simulink model "ASM_Traffic_A11"  (R2026a)
settings: Solver=ode1  StartTime=SIM.tstart.v  StopTime=SIM.tend.v  FixedStep=SIM.StepSize.v
PostLoadFcn:
  | if any(exist('dsrtsu_mdlpostloadfcn', 'file') ~= 0), dsrtsu_mdlpostloadfcn('Execute', bdroot); end
  | try, asm_mdl_postloadfcn(bdroot, 'UpdateModel', 3600); catch, disp(lasterr); end,
InitFcn:
  | , if any(exist('rtifpga_mdlclblib', 'file') ~= 0), rtifpga_mdlclblib('Init', bdroot); end,
  | , if any(exist('dsmpb_private', 'file') ~= 0), dsmpb_private('dsmpb_mdlclblib', 'Init', bdroot); end,
undefined symbols (not defined in the file): _to_, a0b2, ASM_BrakeHydraulics_DemoSystems, ASM_VehicleDynamics_DemoSystems, b98103fe8ad365046cd0, BrakeCircuit, controllerConfig, CPT, Crankshaft, DiscIntNeverNeededParam, dsmsi, FinalDriveAssembly, instance, MDL, ModeSignals, mu, Pos_BrakePedal_Maneuver, rad, RefSignals, s_to_rpm, SIM, SoftECU, Suspension, Tire, Transmission
libraries: ASM_Traffic_lib x135, simulink x98, ASM_Utils_lib x77, ASM_VehicleDynamics_lib x70, ASM_Environment_lib x22, dsmpblib x20, dsmsilib x15, MDLD_Utils_lib x10, ASM_BrakeHydraulics_lib x3, sl_discontinuities x2
(part 14 of 63)

== system ASM_Traffic_A11/Environment/Road/PlantModel ==
  UserInterface : Inport
  In : Inport  Port=2
  AMBIENT : ASM_Environment_lib/Environment/Road/AMBIENT  Tag=ASM_SUBCOMPONENT  Const_temperature=MDL.Environment.Ambient.Const_T  Const_pressure=MDL.Environment.Ambient.Const_p  ASMProperties=struct('Name','AMBIENT','Version','2.0','Library','ASM_Environment_lib')  ASMInstanceName=ambient  ASMInstanceID=1
  ASMSignalCollector : Subsystem
  BASIC_ROADS : ASM_Environment_lib/Environment/Road/BASIC_ROADS  Tag=ASM_SUBCOMPONENT  StepSize=SIM.StepSize  ASMProperties=struct('Name','BASIC_ROADS','Version','13.0','Library','ASM_Environment_lib')  ASMInstanceName=basic_roads  ASMInstanceID=1
  Bus Selector : BusSelector  OutputSignals=ModeSignals.Mode_Road[1NoRoad|2Straight|3Circle|4Road],MdlControl.Reset_VehicleStates[0|1],InitialVehStates.Pos_z_Vehicle_Rel_Init[m],MdlControl.Get_VehPos_Trigger[],Parameters.Curv_Road_Circle[1|m]
  Bus Selector10 : BusSelector  OutputSignals=ExternalModel.s_Preview[m]
  Bus Selector11 : BusSelector  OutputSignals=Slope_BasicRoad[%],Slope_Lateral_BasicRoad[deg],Fric_Coeff_CP_BasicRoad[:][],Sw_Tire_Parameter_Set_CP_BasicRoad[:][1|2|3|4]
  Bus Selector12 : BusSelector  OutputSignals=Sensor_Init_Ready[0Off|1On]
  Bus Selector13 : BusSelector  OutputSignals=ExternalModel.Active_CP_VehDyn_Trailer[]
  Bus Selector14 : BusSelector  OutputSignals=ExternalModel.Pos_CP_FL_CoorSys_E[x;y][m],ExternalModel.Pos_CP_FR_CoorSys_E[x;y][m],ExternalModel.Pos_CP_RL_CoorSys_E[x;y][m],ExternalModel.Pos_CP_RL2_CoorSys_E[x;y][m],ExternalModel.Pos_CP_RR_CoorSys_E[x;y][m],ExternalModel.Pos_CP_RR2_CoorSys_E[x;y][m],ExternalModel.Pos_CP_R2L_CoorSys_E[x;y][m],ExternalModel.Pos_CP_R2L2_CoorSys_E[x;y][m],ExternalModel.Pos_CP_R2R_CoorSys_E[x;y][m],ExternalModel.Pos_CP_R2R2_CoorSys_E[x;y][m],ExternalModel.Pos_CP_FL_Trailer_CoorSys_E[x;y][m],ExternalModel.Pos_CP_FL2_Trailer_CoorSys_E[x;y][m],ExternalModel.Pos_CP_FR_Trailer_CoorSys_E[x;y][m],ExternalModel.Pos_CP_FR2_Trailer_CoorSys_E[x;y][m],ExternalModel.Pos_CP_RL_Trailer_CoorSys_E[x;y][m],ExternalModel.Pos_CP_RL2_Trailer_CoorSys_E[x;y][m],ExternalModel.Pos_CP_RR_Trailer_CoorSys_E[x;y][m],ExternalModel.Pos_CP_RR2_Trailer_CoorSys_E[x;y][m],ExternalModel.Pos_CP_R2L_Trailer_CoorSys_E[x;y][m],ExternalModel.Pos_CP_R2L2_Trailer_CoorSys_E[x;y][m],ExternalModel.Pos_CP_R2R_Trailer_CoorSys_E[x;y][m],ExternalModel.Pos_CP_R2R2_Trailer_CoorSys_E[x;y][m],ExternalModel.Pos_CP_Front_CoorSys_E[x;y][m],ExternalModel.Pos_CP_Rear_CoorSys_E[x;y][m]  OutputAsBus=on
  Bus Selector15 : BusSelector  OutputSignals=ExternalModel.Angle_Vehicle_CoorSys_E[x;y;z][deg],ExternalModel.Pos_Vehicle_CoorSys_E[x;y;z][m]
  Bus Selector2 : BusSelector  OutputSignals=Sw_BasicRoad,Sw_RoadSelect[1_6]
  Bus Selector3 : BusSelector  OutputSignals=Route_Id_Fellows_Ref_Scheduler[],Direction_Fellows_Ref_Scheduler[-1|1],s_Fellows_Ref_Scheduler[m],d_Fellows_Ref_Scheduler[m],LaneIdx_Fellows_Ref_Scheduler[],RelativeLane_Mode_Fellows[0CenterLane|1PreferredLane],v_Lat_Fellows_Ref_Scheduler[m|s],ForceToRoad_Fellows_Ref_Scheduler[0|1],Flag_FellowUsed[0|1],Dist_Def_Trf[]
  Bus Selector4 : BusSelector  OutputSignals=Maneuver.Plant.ManeuverScheduler,Interface_In,Traffic.Plant.Traffic_Signals_toEnvironment,Sensors.Plant.Sensors_Common
  Bus Selector5 : BusSelector  OutputSignals=MdlControl.RoadControl[],InitialVehStates.Pos_z_Vehicle_Rel_Init[m],InitialVehStates.Angle_Yaw_Vehicle_Rel_Init[deg],InitialVehStates.Route_Id_Init[],InitialVehStates.Route_Direction_Init[],InitialVehStates.s_Vehicle_Init[m],InitialVehStates.d_Vehicle_Init[m],InitialVehStates.LaneIdx_Vehicle_Init[],RefSignals.d_Maneuver[m],RefSignals.LaneIdx_Maneuver[],ModeSignals.Mode_RelativeLane[0CenterLane|1PreferredLane],Parameters.v_Lat[m|s],ModeSignals.Mode_ForceToRoad[1Off|2On],RefSignals.Dist_Def_Maneuver[]
  Bus Selector7 : BusSelector  OutputSignals=ExternalModel.RotationMatrix_V_to_E[1x9]
  Bus Selector8 : BusSelector  OutputSignals=ExternalModel.v_x_Vehicle_CoG[km|h]
  Bus Selector9 : BusSelector  OutputSignals=Control.Interface_Mode[0Off|1ObjOnly|2ObjAndLanes],Control.Quadrant_Def_Mode[1Internal|2External],Control.Quadrant_Dim_x[m],Control.Quadrant_Dim_y[m]
  Const_4Road : Constant  Value=4
  Constant1 : Constant  Value=0
  Constant2 : Constant  Value=0
  Customize_UserSignals : Subsystem
  Demux : Demux  Outputs=3
  Demux1 : Demux  Outputs=3
  GPS_POSITION : ASM_Environment_lib/Environment/Road/GPS_POSITION  Tag=ASM_SUBCOMPONENT  ASMProperties=struct('Name','GPS_POSITION','Version','3.0','Library','ASM_Environment_lib')  ASMInstanceName=GPS_Position  ASMInstanceID=1
  Goto Tag Visibility : GotoTagVisibility  GotoTag=ASMBUS_Environment_BasicRoads
  Goto Tag Visibility1 : GotoTagVisibility  GotoTag=ASMBUS_Environment_StandardRoad
  Goto Tag Visibility2 : GotoTagVisibility  GotoTag=ASMBUS_Environment_LaneSensor_Dynamic_Parameters
  Goto Tag Visibility3 : GotoTagVisibility  GotoTag=ASMBUS_Environment_LaneSensor_Dynamic_Output
  Goto Tag Visibility4 : GotoTagVisibility  GotoTag=ASMBUS_Environment_Customized_UserSignals
  Goto Tag Visibility5 : GotoTagVisibility  GotoTag=ASMBUS_Environment_PosVehGPS
  Goto Tag Visibility6 : GotoTagVisibility  GotoTag=ASMBUS_Environment_Ambient
  Goto Tag Visibility7 : GotoTagVisibility  GotoTag=ASMBUS_Environment_Lane_Network
  LANESENSOR_DYNAMIC_OUTPUT : ASM_Environment_lib/Environment/Road/LANESENSOR_DYNAMIC_OUTPUT  Const_SensorPoints_OutputDimension=MDL.Environment.Road.LaneSensorDynamic_Output.Const_SensorPoints_OutputDimension  Const_MeasPoints_OutputDimension=MDL.Environment.Road.LaneSensorDynamic_Output.Const_MeasPoints_OutputDimension  Const_LanesLeft_OutputDimension=MDL.Environment.Road.LaneSensorDynamic_Output.Const_LanesLeft_OutputDimension  Const_LanesRight_OutputDimension=MDL.Environment.Road.LaneSensorDynamic_Output.Const_LanesRight_OutputDimension  ASMProperties=struct('Name','LANESENSOR_DYNAMIC_OUTPUT','Version','2.0','Library','ASM_Environment_lib')  ASMInstanceName=lanesensor_dynamic_output  ASMInstanceID=1
  LANESENSOR_DYNAMIC_PARAMETERS : ASM_Environment_lib/Environment/Road/LANESENSOR_DYNAMIC_PARAMETERS  Tag=ASM_SUBCOMPONENT  Sw_LaneSensor_Enable=MDL.Environment.Road.LaneSensorDynamic_Parameters.Sw_LaneSensor_Enable  Const_Dist_LaneSensor=MDL.Environment.Road.LaneSensorDynamic_Parameters.Const_Dist_LaneSensor  Sw_LaneSensor_Border_Mode=MDL.Environment.Road.LaneSensorDynamic_Parameters.Sw_LaneSensor_Border_Mode  Sw_LaneSensor_Junction_Enable=MDL.Environment.Road.LaneSensorDynamic_Parameters.Sw_LaneSensor_Junction_Enable  Const_NumLanes_Left=MDL.Environment.Road.LaneSensorDynamic_Parameters.Const_NumLanes_Left  Const_NumLanes_Right=MDL.Environment.Road.LaneSensorDynamic_Parameters.Const_NumLanes_Right  Sw_LaneSensor_MeasPoint_Enable=MDL.Environment.Road.LaneSensorDynamic_Parameters.Sw_LaneSensor_MeasPoint_Enable  Const_Pos_MeasPoint_1=MDL.Environment.Road.LaneSensorDynamic_Parameters.Const_Pos_MeasPoint_1  Const_Pos_MeasPoint_2=MDL.Environment.Road.LaneSensorDynamic_Parameters.Const_Pos_MeasPoint_2  Const_Pos_MeasPoint_3=MDL.Environment.Road.LaneSensorDynamic_Parameters.Const_Pos_MeasPoint_3  Const_Pos_MeasPoint_4=MDL.Environment.Road.LaneSensorDynamic_Parameters.Const_Pos_MeasPoint_4  ASMProperties=struct('Name','LANESENSOR_DYNAMIC_PARAMETERS','Version','1.0','Library','ASM_Environment_lib')  ASMInstanceName=lanesensor_dynamic_parameters  ASMInstanceID=1
  LANE_NETWORK : ASM_Environment_lib/Environment/Road/LANE_NETWORK  Tag=ASM_SUBCOMPONENT  LaneNetwork_ModelDesk=MDL.Environment.LaneNetwork.LaneNetwork_ModelDesk  LaneNetwork_2=MDL.Environment.LaneNetwork.LaneNetwork_2  LaneNetwork_3=MDL.Environment.LaneNetwork.LaneNetwork_3  LaneNetwork_4=MDL.Environment.LaneNetwork.LaneNetwork_4  LaneNetwork_5=MDL.Environment.LaneNetwork.LaneNetwork_5  LaneNetwork_6=MDL.Environment.LaneNetwork.LaneNetwork_6  Const_Quad_Dim_x=MDL.Environment.LaneNetwork.Const_Section_Dim_x  Const_Quad_Dim_y=MDL.Environment.LaneNetwork.Const_Section_Dim_y  Const_Max_Num_Lb_Quad=MDL.Environment.LaneNetwork.Const_Max_Num_Lb_Per_Section  Const_Max_Num_Pnts_Load=MDL.Environment.LaneNetwork.Const_Max_Num_Pnts_Per_Step  Const_Max_Num_Lanes_Load=MDL.Environment.LaneNetwork.Const_Max_Num_Lanes_Per_Step  Const_Max_Num_Lb_Free=MDL.Environment.LaneNetwork.Const_Max_Num_Lb_Free_Per_Step  Const_Max_Num_Lanes_Free=MDL.Environment.LaneNetwork.Const_Max_Num_Lanes_Free_Per_Step  ASMProperties=struct('Name','LANE_NETWORK','Version','5.0','Library','ASM_Environment_lib')  ASMInstanceName=lane_network  ASMInstanceID=1
  Mux : Mux  Inputs=2
  Mux1 : Mux  Inputs=2
  NoRoad : RelationalOperator  Operator===  OutDataTypeStr=boolean  InputSameDT=off
  Pos_CP_CoorsSys_E[:][x;y][m] : Subsystem
  Product1 : Product  RndMeth=Zero
  Product8 : Product  RndMeth=Zero
  ROAD : ASM_Environment_lib/Environment/Road/ROAD  Tag=ASM_SUBCOMPONENT  Road_ModelDesk=MDL.Environment.Road.Road_ModelDesk  Road_2=MDL.Environment.Road.Road_2  Road_3=MDL.Environment.Road.Road_3  Road_4=MDL.Environment.Road.Road_4  Road_5=MDL.Environment.Road.Road_5  Road_6=MDL.Environment.Road.Road_6  StepSize=SIM.StepSize  ASMProperties=struct('Name','ROAD','Version','32.0','Library','ASM_Environment_lib')  ASMInstanceName=road  ASMInstanceID=1
  Reload_Trigger : Subsystem
  Sat_RoadMode : Saturate  UpperLimit=4  LowerLimit=1
  Terminator{,1..19} (20 alike) : Terminator
  "[1x9]to[3x3]" : Reshape  OutputDimensionality=Customize  OutputDimensions=[3,3]
  ones26 : Constant  Value=ones(1,26)  OutDataTypeStr=double
  zero : Constant  Value=0
  ASMSignalBus : Outport  VectorParamsAs1DForOutWhenUnconnected=off
  tag scope: ASMBUS_Environment_Ambient=scoped, ASMBUS_Environment_BasicRoads=scoped, ASMBUS_Environment_Customized_UserSignals=scoped, ASMBUS_Environment_LaneSensor_Dynamic_Output=scoped, ASMBUS_Environment_LaneSensor_Dynamic_Parameters=scoped, ASMBUS_Environment_Lane_Network=scoped, ASMBUS_Environment_PosVehGPS=scoped, ASMBUS_Environment_StandardRoad=scoped
  wires:
  Bus Selector12/1 -> Reload_Trigger/1(Init_External_Additional[0Off|1On])  "<Sensor_Init_Ready[0Off|1On]>"
  Bus Selector4/4 -> Bus Selector12/1  "<Sensors_Common>"
  LANESENSOR_DYNAMIC_OUTPUT/2 -> Terminator7/1
  GPS_POSITION/2 -> Terminator6/1
  ROAD/10 -> Terminator3/1
  ROAD/8 -> Terminator2/1
  ROAD/6 -> Terminator1/1
  LANESENSOR_DYNAMIC_PARAMETERS/1 -> [ASMBUS_Environment_LaneSensor_Dynamic_Parameters]
  Bus Selector4/3 -> Bus Selector3/1, Bus Selector9/1  "<Traffic_Signals_toEnvironment>"
  GPS_POSITION/1 -> [ASMBUS_Environment_PosVehGPS]
  AMBIENT/2 -> Terminator4/1  "T_Ambient[degC]"
  Bus Selector10/1 -> Mux/2, BASIC_ROADS/6  "<s_Preview[m]>"
  Bus Selector4/1 -> Bus Selector/1, Bus Selector5/1  "<ManeuverScheduler>"
  Demux1/3 -> BASIC_ROADS/7, ROAD/19
  ROAD/4 -> Terminator11/1
  Bus Selector3/10 -> ROAD/32  "<Dist_Def_Trf[]>"
  In/1 -> Bus Selector4/1
  Bus Selector/2 -> BASIC_ROADS/2  "<Reset_VehicleStates[0|1]>"
  Bus Selector11/2 -> BASIC_ROADS/13  "<Slope_Lateral_BasicRoad[deg]>"
  Bus Selector7/1 -> "[1x9]to[3x3]"/1  "<RotationMatrix_V_to_E[1x9]>"
  Bus Selector9/1 -> LANE_NETWORK/3, Reload_Trigger/2(Interface_Mode[0Off|1ObjectsOnly|2ObjectsAndLanes])  "<Interface_Mode[0Off|1ObjOnly|2ObjAndLanes]>"
  Bus Selector11/4 -> BASIC_ROADS/15  "<Sw_Tire_Parameter_Set_CP_BasicRoad[:][1|2|3|4]>"
  Mux1/1 -> LANE_NETWORK/5
  Bus Selector5/12 -> ROAD/13  "<v_Lat[m|s]>"
  Bus Selector2/2 -> LANE_NETWORK/1, ROAD/1  "<Sw_RoadSelect[1_6]>"
  Bus Selector9/3 -> Mux1/1  "<Quadrant_Dim_x[m]>"
  Demux/2 -> BASIC_ROADS/9, LANESENSOR_DYNAMIC_PARAMETERS/2, GPS_POSITION/3, ROAD/18
  Bus Selector5/8 -> ROAD/9  "<LaneIdx_Vehicle_Init[]>"
  LANESENSOR_DYNAMIC_PARAMETERS/2 -> ROAD/33
  Bus Selector9/4 -> Mux1/2  "<Quadrant_Dim_y[m]>"
  ASMSignalCollector/1(Road_Signals) -> ASMSignalBus/1  "Plant"
  Bus Selector11/3 -> BASIC_ROADS/14  "<Fric_Coeff_CP_BasicRoad[:][]>"
  LANESENSOR_DYNAMIC_PARAMETERS/8 -> ROAD/39
  LANESENSOR_DYNAMIC_PARAMETERS/3 -> ROAD/34
  Bus Selector3/6 -> ROAD/28  "<RelativeLane_Mode_Fellows[0CenterLane|1PreferredLane]>"
  LANESENSOR_DYNAMIC_OUTPUT/1 -> [ASMBUS_Environment_LaneSensor_Dynamic_Output]
  LANESENSOR_DYNAMIC_PARAMETERS/7 -> ROAD/38
  Bus Selector3/7 -> ROAD/29  "<v_Lat_Fellows_Ref_Scheduler[m|s]>"
  Bus Selector2/1 -> Bus Selector11/1  "<Sw_BasicRoad>"
  Product1/1 -> ROAD/10
  Bus Selector3/9 -> ROAD/31  "<Flag_FellowUsed[0|1]>"
  Bus Selector5/14 -> ROAD/15  "<Dist_Def_Maneuver[]>"
  Bus Selector3/3 -> ROAD/25  "<s_Fellows_Ref_Scheduler[m]>"
  Product8/1 -> ROAD/11
  Bus Selector5/5 -> ROAD/6  "<Route_Direction_Init[]>"
  Bus Selector3/2 -> ROAD/24  "<Direction_Fellows_Ref_Scheduler[-1|1]>"
  Mux/1 -> ROAD/16
  Reload_Trigger/1(Ctrl_Reload[]) -> LANE_NETWORK/2
  ROAD/5 -> Terminator12/1
  Bus Selector/1 -> BASIC_ROADS/1, Sat_RoadMode/1  "<Mode_Road[1NoRoad|2Straight|3Circle|4Road]>"
  Bus Selector9/2 -> LANE_NETWORK/4  "<Quadrant_Def_Mode[1Internal|2External]>"
  BASIC_ROADS/5 -> Terminator15/1
  Bus Selector3/8 -> ROAD/30  "<ForceToRoad_Fellows_Ref_Scheduler[0|1]>"
  LANESENSOR_DYNAMIC_PARAMETERS/5 -> ROAD/36
  zero/1 -> Mux/1
  Const_4Road/1 -> NoRoad/2
  Bus Selector/3 -> BASIC_ROADS/3  "<Pos_z_Vehicle_Rel_Init[m]>"
  ones26/1 -> Product1/1, Product8/1
  BASIC_ROADS/1 -> [ASMBUS_Environment_BasicRoads]
  ROAD/3 -> Terminator10/1
  Sat_RoadMode/1 -> NoRoad/1
  ROAD/11 -> LANESENSOR_DYNAMIC_OUTPUT/1
  ROAD/7 -> Terminator/1
  ROAD/9 -> Customize_UserSignals/1(UserSignals_In)
  Bus Selector3/4 -> ROAD/26  "<d_Fellows_Ref_Scheduler[m]>"
  Bus Selector5/1 -> ROAD/2  "<RoadControl[]>"
  Bus Selector/5 -> BASIC_ROADS/5  "<Curv_Road_Circle[1|m]>"
  Bus Selector5/4 -> ROAD/5  "<Route_Id_Init[]>"
  Bus Selector/4 -> BASIC_ROADS/4  "<Get_VehPos_Trigger[]>"
  Bus Selector11/1 -> BASIC_ROADS/12  "<Slope_BasicRoad[%]>"
  Constant2/1 -> ROAD/22
  Bus Selector5/10 -> Product8/2  "<LaneIdx_Maneuver[]>"
  BASIC_ROADS/3 -> Terminator13/1
  Demux/1 -> ROAD/17, LANESENSOR_DYNAMIC_PARAMETERS/1, GPS_POSITION/2, BASIC_ROADS/8
  BASIC_ROADS/4 -> Terminator14/1
  LANESENSOR_DYNAMIC_PARAMETERS/4 -> ROAD/35
  Bus Selector5/11 -> ROAD/12  "<Mode_RelativeLane[0CenterLane|1PreferredLane]>"
  AMBIENT/3 -> Terminator16/1  "p_Ambient[Pa]"
  Bus Selector5/6 -> ROAD/7  "<s_Vehicle_Init[m]>"
  Constant1/1 -> ROAD/21
  Bus Selector5/7 -> ROAD/8  "<d_Vehicle_Init[m]>"
  LANESENSOR_DYNAMIC_PARAMETERS/6 -> ROAD/37
  NoRoad/1 -> ASMSignalCollector/1(SwitchRoad[0BasicRoad|1StandardRoad])
  Bus Selector3/1 -> ROAD/23  "<Route_Id_Fellows_Ref_Scheduler[]>"
  LANE_NETWORK/1 -> [ASMBUS_Environment_Lane_Network]
  ROAD/1 -> [ASMBUS_Environment_StandardRoad]
  Customize_UserSignals/1(ASMSignalBus) -> [ASMBUS_Environment_Customized_UserSignals]
  Bus Selector5/3 -> ROAD/4  "<Angle_Yaw_Vehicle_Rel_Init[deg]>"
  Bus Selector5/2 -> ROAD/3  "<Pos_z_Vehicle_Rel_Init[m]>"
  Bus Selector5/13 -> ROAD/14  "<Mode_ForceToRoad[1Off|2On]>"
  Bus Selector5/9 -> Product1/2  "<d_Maneuver[m]>"
  AMBIENT/1 -> [ASMBUS_Environment_Ambient]
  UserInterface/1 -> Bus Selector2/1
  Customize_UserSignals/2(UserSignals_Customized) -> GPS_POSITION/1
  ROAD/2 -> Terminator5/1
  BASIC_ROADS/2 -> Terminator8/1
  Bus Selector3/5 -> ROAD/27  "<LaneIdx_Fellows_Ref_Scheduler[]>"
  "[1x9]to[3x3]"/1 -> LANESENSOR_DYNAMIC_PARAMETERS/3
  LANE_NETWORK/2 -> Terminator9/1  "LaneNetwork_Data[]"
  Bus Selector4/2 -> Bus Selector8/1, Bus Selector10/1, Bus Selector15/1, Bus Selector14/1, Bus Selector13/1, Bus Selector7/1  "<Interface_In>"
  Bus Selector14/1 -> Pos_CP_CoorsSys_E[:][x;y][m]/1(Pos_CP[x;y][m])
  Bus Selector13/1 -> Pos_CP_CoorsSys_E[:][x;y][m]/2(Active_CP_VehDyn_Trailer[])  "<Active_CP_VehDyn_Trailer[]>"
  Pos_CP_CoorsSys_E[:][x;y][m]/1(Pos_CP_CoorsSys_E[:][x;y][m]) -> ROAD/20, BASIC_ROADS/10
  Bus Selector8/1 -> BASIC_ROADS/11  "<v_x_Vehicle_CoG[km|h]>"
  Demux/3 -> Terminator17/1
  Bus Selector15/2 -> Demux/1  "<Pos_Vehicle_CoorSys_E[x;y;z][m]>"
  Bus Selector15/1 -> Demux1/1  "<Angle_Vehicle_CoorSys_E[x;y;z][deg]>"
  Demux1/1 -> Terminator18/1
  Demux1/2 -> Terminator19/1

== system ASM_Traffic_A11/Environment/Road/UserInterface ==
  note: Road
  Interface_In : Inport
  In : Inport  Port=2
  ASMSignalBus_Plant : Subsystem
  DISP_Plant : Subsystem
  PAR_Plant : Subsystem
  Out : Outport  VectorParamsAs1DForOutWhenUnconnected=off
  wires:
  PAR_Plant/1(Out) -> Out/1
  Interface_In/1 -> PAR_Plant/1(Interface_In)
  In/1 -> ASMSignalBus_Plant/1(In), DISP_Plant/1(In)

== system ASM_Traffic_A11/Environment/Sensors/PlantModel ==
  UserInterface : Inport
  In : Inport  Port=2
  ASMSignalCollector : Subsystem
  Bus Selector7 : BusSelector  OutputSignals=Traffic,Interface_In,Road,Maneuver,Road.UserInterface.Objects_DataStreams[]
  Collision_Sensor : Subsystem
  Line_Sensor : Subsystem
  Object_Sensor_2D : Subsystem
  Object_Sensor_3D : Subsystem
  SensorsGotoTagVisiblity : GotoTagVisibility  GotoTag=ASMBUS_Environment_Trafffic_Sensors_Object_Sensor_3D
  SensorsGotoTagVisiblity1 : GotoTagVisibility  GotoTag=ASMBUS_Environment_Traffic_Sensors_Object_Sensor_2D
  SensorsGotoTagVisiblity2 : GotoTagVisibility  GotoTag=ASMBUS_Environment_Traffic_Sensors_Traffic_Sign_Sensor_dyn
  SensorsGotoTagVisiblity3 : GotoTagVisibility  GotoTag=ASMBUS_Environment_Traffic_Sensors_Line_Sensor
  SensorsGotoTagVisiblity4 : GotoTagVisibility  GotoTag=ASMBUS_Environment_Traffic_Sensors_Collision_Sensor
  SensorsGotoTagVisiblity5 : GotoTagVisibility  GotoTag=ASMBUS_Environment_Traffic_Sensors_Common
  Sensors_Common_Signals : Subsystem
  Terminator{,1..5} (6 alike) : Terminator
  Traffic_Sign_Sensor : Subsystem
  ASMSignalBus : Outport  VectorParamsAs1DForOutWhenUnconnected=off
  tag scope: ASMBUS_Environment_Traffic_Sensors_Common=scoped
  wires:
  In/1 -> Sensors_Common_Signals/1(In), Bus Selector7/1
  Sensors_Common_Signals/1(ASMSignalBus) -> [ASMBUS_Environment_Traffic_Sensors_Common]
  Object_Sensor_3D/2(Init_Ready[0Off|1On]) -> Object_Sensor_2D/1(Enable_Init[0Off|1On])
  Sensors_Common_Signals/4(Enable_Sensor_Scheduling[0Off|1On]) -> Line_Sensor/1(Enable[0Off|1On])
  Object_Sensor_2D/2(Init_Ready[0Off|1On]) -> Sensors_Common_Signals/2(Init_Ready[0Off|1On]), Collision_Sensor/1(Enable_Init[0Off|1On])
  Sensors_Common_Signals/2(Enable_Init[0Off|1On]) -> Object_Sensor_3D/1(Enable_Init[0Off|1On])
  Sensors_Common_Signals/3(Enable_Sensor_Scheduling_By_Init_Ready[0Off|1On]) -> Object_Sensor_2D/2(Enable[0Off|1On]), Collision_Sensor/2(Enable[0Off|1On]), Object_Sensor_3D/2(Enable[0Off|1On])
  Object_Sensor_3D/1(Sensor_Signals) -> Terminator5/1  "Object_Sensor_3D"
  Object_Sensor_2D/1(Sensor_Signals) -> Terminator1/1  "Object_Sensor_2D"
  Traffic_Sign_Sensor/1(Sensor_Signals) -> Terminator2/1  "Traffic_Sign_Sensor"
  Line_Sensor/1(Sensor_Signals) -> Terminator3/1  "Line_Sensor"
  Collision_Sensor/1(Sensor_Signals) -> Terminator4/1  "Collision_Sensor"
  ASMSignalCollector/1(Sensors) -> ASMSignalBus/1  "Plant"
  UserInterface/1 -> Terminator/1
  Bus Selector7/5 -> Traffic_Sign_Sensor/4(Objects_DataStream_Signals)  "<Objects_DataStreams[]>"
  Bus Selector7/4 -> Collision_Sensor/6(Maneuver_Signals), Line_Sensor/4(Maneuver_Signals)  "<Maneuver>"
  Bus Selector7/3 -> Collision_Sensor/5(Road_Signals), Line_Sensor/3(Road_Signals), Traffic_Sign_Sensor/3(Road_Signals), Object_Sensor_2D/5(Road_Signals), Object_Sensor_3D/5(Road_Signals)  "<Road>"
  Bus Selector7/1 -> Collision_Sensor/3(Traffic_Signals), Traffic_Sign_Sensor/2(Traffic_Signals), Object_Sensor_2D/3(Traffic_Signals), Object_Sensor_3D/3(Traffic_Signals)  "<Traffic>"
  Bus Selector7/2 -> Collision_Sensor/4(Interface_In), Line_Sensor/2(Interface_In), Traffic_Sign_Sensor/1(Interface_In), Object_Sensor_2D/4(Interface_In), Object_Sensor_3D/4(Interface_In)  "<Interface_In>"
  Sensors_Common_Signals/5(Sensor_Time_Base[s]) -> Object_Sensor_3D/6(Sensor_Time_Base[s])

== system ASM_Traffic_A11/Environment/Sensors/UserInterface ==
  note: Sensors
  In : Inport
  ASMSignalBus_Plant : Subsystem
  DISP_Plant : Subsystem
  PAR_Plant : Subsystem
  Out : Outport  VectorParamsAs1DForOutWhenUnconnected=off
  wires:
  PAR_Plant/1(Out) -> Out/1
  In/1 -> ASMSignalBus_Plant/1(In), PAR_Plant/1(In), DISP_Plant/1(In)

== system ASM_Traffic_A11/Environment/SignalInterface/ASMSignalInterface ==
  ASMSignalBus : Inport
  Enable : EnablePort
  signal_structure : Subsystem
  wires:
  ASMSignalBus/1 -> signal_structure/1(ASMSignalBus)

== system ASM_Traffic_A11/Environment/SignalInterface/ExternalOutports ==
  In1 : Inport
  Enable : EnablePort
  Environment : dsmpblib/Data Outport  Tag=ASM_MPB  Priority=-10000
      settings: SourceProductName=dSPACE Model Interface Package for Simulink (MIPS)
  Select_Outport_Signals : Subsystem
  wires:
  In1/1 -> Select_Outport_Signals/1(ASMSignalBus)
  Select_Outport_Signals/5(Sensors) -> Environment/5
  Select_Outport_Signals/4(GroundTruth) -> Environment/4
  Select_Outport_Signals/3(Traffic) -> Environment/3
  Select_Outport_Signals/2(Road) -> Environment/2
  Select_Outport_Signals/1(Maneuver) -> Environment/1

== system ASM_Traffic_A11/Environment/SignalInterface/Reduce_ASMSignalBus ==
  ASMSignalBus : Inport
  Bus Creator : BusCreator  Inputs=5
  Bus Creator1 : BusCreator  Inputs=8
  Bus Creator2 : BusCreator  Inputs=8
  Bus Creator3 : BusCreator  Inputs=6
  Bus Creator4 : BusCreator  Inputs=5
  Bus Selector : BusSelector  OutputSignals=Maneuver,Road,Traffic,GroundTruth,Sensors
  Bus Selector1 : BusSelector  OutputSignals=Parameter,SensorIndex,Info,SensorOutput,SensorTimeStamp,RadarEffects,CustomPoints,ObjectData
  Bus Selector2 : BusSelector  OutputSignals=Parameter,SensorIndex,Info,SensorOutput,SensorTimeStamp,RadarEffects,CustomPoints,ObjectData
  Bus Selector3 : BusSelector  OutputSignals=Parameters,SensorIndex,SensorStatus,SensorOutput,Info,ObjectData
  Bus Selector4 : BusSelector  OutputSignals=Collision_Sensor,TrafficSign_Sensor_Dyn,Object_Sensor_3D.Sensor_1_Front_Long,Object_Sensor_3D.Sensor_2_Front_Mid,Object_Sensor_2D.Sensor_1_Front
  ASMSignalBus_Reduced : Outport  VectorParamsAs1DForOutWhenUnconnected=off
  wires:
  Bus Selector3/6 -> Bus Creator3/6  "<ObjectData>"
  Bus Selector3/5 -> Bus Creator3/5  "<Info>"
  Bus Selector3/4 -> Bus Creator3/4  "<SensorOutput>"
  Bus Selector3/3 -> Bus Creator3/3  "<SensorStatus>"
  Bus Selector3/2 -> Bus Creator3/2  "<SensorIndex>"
  Bus Selector3/1 -> Bus Creator3/1  "<Parameters>"
  Bus Creator3/1 -> Bus Creator4/5  "Object_Sensor_2D_1"
  Bus Selector4/5 -> Bus Selector3/1  "<Sensor_1_Front>"
  Bus Selector4/4 -> Bus Selector2/1  "<Sensor_2_Front_Mid>"
  Bus Selector2/1 -> Bus Creator2/1  "<Parameter>"
  Bus Selector2/2 -> Bus Creator2/2  "<SensorIndex>"
  Bus Selector2/3 -> Bus Creator2/3  "<Info>"
  Bus Selector2/4 -> Bus Creator2/4  "<SensorOutput>"
  Bus Selector2/5 -> Bus Creator2/5  "<SensorTimeStamp>"
  Bus Selector2/6 -> Bus Creator2/6  "<RadarEffects>"
  Bus Selector2/7 -> Bus Creator2/7  "<CustomPoints>"
  Bus Selector2/8 -> Bus Creator2/8  "<ObjectData>"
  Bus Creator2/1 -> Bus Creator4/4  "Object_Sensor_3D_2"
  Bus Creator1/1 -> Bus Creator4/3  "Object_Sensor_3D_1"
  Bus Selector1/8 -> Bus Creator1/8  "<ObjectData>"
  Bus Selector1/7 -> Bus Creator1/7  "<CustomPoints>"
  Bus Selector1/6 -> Bus Creator1/6  "<RadarEffects>"
  Bus Selector1/5 -> Bus Creator1/5  "<SensorTimeStamp>"
  Bus Selector1/4 -> Bus Creator1/4  "<SensorOutput>"
  Bus Selector1/3 -> Bus Creator1/3  "<Info>"
  Bus Selector1/2 -> Bus Creator1/2  "<SensorIndex>"
  Bus Selector1/1 -> Bus Creator1/1  "<Parameter>"
  Bus Selector4/3 -> Bus Selector1/1  "<Sensor_1_Front_Long>"
  Bus Selector4/2 -> Bus Creator4/2  "<TrafficSign_Sensor_Dyn>"
  Bus Selector/2 -> Bus Creator/2  "<Road>"
  Bus Selector/3 -> Bus Creator/3  "<Traffic>"
  Bus Creator/1 -> ASMSignalBus_Reduced/1
  Bus Selector/1 -> Bus Creator/1  "<Maneuver>"
  ASMSignalBus/1 -> Bus Selector/1
  Bus Selector/4 -> Bus Creator/4  "<GroundTruth>"
  Bus Selector/5 -> Bus Selector4/1  "<Sensors>"
  Bus Selector4/1 -> Bus Creator4/1  "<Collision_Sensor>"
  Bus Creator4/1 -> Bus Creator/5  "Sensors"

== system ASM_Traffic_A11/Environment/Traffic/PlantModel ==
  UserInterface : Inport
  In : Inport  Port=2
  Bus Creator2 : BusCreator  Inputs=4
  Bus Selector1 : BusSelector  OutputSignals=FellowSignalLabels
  Bus Selector16 : BusSelector  OutputSignals=Road,Maneuver,Interface_In,Traffic.Plant.ObjectParameters,Road.UserInterface.Objects_DataStreams[],Traffic,GroundTruth,Sensors
  FellowMovement : Subsystem
  Merge_Signals_toEnvironment : Subsystem
  ObjectParameters : Subsystem
  V2X : Subsystem
  ASMSignalBus : Outport  VectorParamsAs1DForOutWhenUnconnected=off
  wires:
  ObjectParameters/1(Objects_Signals) -> Bus Creator2/3
  Bus Selector1/1 -> Bus Creator2/2  "<FellowSignalLabels>"
  FellowMovement/1(FellowMovement_Signals) -> Bus Selector1/1, Merge_Signals_toEnvironment/1(Traffic_Signals)
  Bus Selector16/7 -> Merge_Signals_toEnvironment/2(GroundTruth_Interface)  "<GroundTruth>"
  Bus Creator2/1 -> ASMSignalBus/1  "Plant"
  Bus Selector16/5 -> FellowMovement/6(Object_DataStreams)  "<Objects_DataStreams[]>"
  In/1 -> Bus Selector16/1
  Bus Selector16/3 -> FellowMovement/4(Interface_In)  "<Interface_In>"
  UserInterface/1 -> V2X/3(UserInterface), FellowMovement/1(UserInterface)
  Merge_Signals_toEnvironment/1(Signals_toEnvironment) -> Bus Creator2/1
  Bus Selector16/2 -> V2X/2(Maneuver_Signals), ObjectParameters/2(Maneuver_Signals), FellowMovement/3(Maneuver_Signals)  "<Maneuver>"
  Bus Selector16/1 -> ObjectParameters/1(Road_Signals), V2X/1(Road_Signals), FellowMovement/2(Road_Signals)  "<Road>"
  Bus Selector16/4 -> FellowMovement/5(ObjectParameters_Signals)  "<ObjectParameters>"
  V2X/1(V2X_Signals) -> Bus Creator2/4
  Bus Selector16/6 -> FellowMovement/7(Traffic_Signals)  "<Traffic>"
  Bus Selector16/8 -> ObjectParameters/3(Sensor_Signals)  "<Sensors>"

== system ASM_Traffic_A11/Environment/Traffic/UserInterface ==
  note: Traffic
  In : Inport
  ASMSignalBus_Plant : Subsystem
  DISP_Plant : Subsystem
  PAR_Plant : Subsystem
  Out : Outport  VectorParamsAs1DForOutWhenUnconnected=off
  wires:
  PAR_Plant/1(Out) -> Out/1
  In/1 -> ASMSignalBus_Plant/1(In), DISP_Plant/1(In)

== system ASM_Traffic_A11/VehicleDynamics/Control/SoftECU_Brake ==
  note: -------------
  note: Control
  note: -------------
  note: -------------
  note: -------------
  note: Inport colors:
  note: User Interface
  note: Plant
  note: External Signals
  UserInterface : Inport
  Interface_In : Inport  Port=2
  Plant : Inport  Port=3
  Brake_Topology_Switch : Subsystem
  Bus Creator : BusCreator  Inputs=5
  Bus Selector1 : BusSelector  OutputSignals=ExternalModel.Enable_Trq_Brake_Extern[0|1],ExternalModel.Trq_Brake_Request_Extern[Nm],ExternalModel.Trq_Request_Brake[Nm]
  Bus Selector10 : BusSelector  OutputSignals=ExternalModel.Vehicle_Topology[-2|-1|0|2],ExternalModel.Trq_Eff_Engine[Nm],ExternalModel.Trq_EM_Front[Nm]
  Bus Selector2 : BusSelector  OutputSignals=VehicleDynamics.Brake.BrakeDisc.Const_BrakeDiscFactor.Const_BrakeDiscFactor_FL[m3],VehicleDynamics.Brake.BrakeDisc.Const_BrakeDiscFactor.Const_BrakeDiscFactor_FR[m3],VehicleDynamics.Brake.BrakeDisc.Const_BrakeDiscFactor.Const_BrakeDiscFactor_RL[m3],VehicleDynamics.Brake.BrakeDisc.Const_BrakeDiscFactor.Const_BrakeDiscFactor_RR[m3],VehicleDynamics.Brake.MasterBrakeCylinder.ActiveBrakeCylinder.p[bar],VehicleDynamics.VehicleMovement.Velocities.Vehicle.Linear.v_Vehicle_CoG[x;y;z][km|h].v_x_Vehicle_CoG[km|h],VehicleDynamics.VehicleMovement.Velocities.Vehicle.Linear.v_Vehicle_CoG[x;y;z][km|h].v_y_Vehicle_CoG[km|h],VehicleDynamics.VehicleMovement.Accelerations.VehicleCoG.Linear.a_Vehicle_CoG[x;y;z][m|s2].a_y_Vehicle_CoG[m|s2],VehicleDynamics.VehicleMovement.Velocities.Vehicle.Angular.w_Vehicle_CoG[x;y;z][deg|s].YawRate_Vehicle_CoG[deg|s],VehicleDynamics.Wheel.WheelSpeed2.omega_Wheel[FL;FR;RL;RR][rad|s],VehicleDynamics.Steering.Angle_SteeringWheel[deg],VehicleDynamics.Steering.i_Steering_Mean[],VehicleDynamics.Suspension.SuspensionRear.RelativePositionRear.Pos_Wheel[RL;RR][x;y;z][m].Pos_RL_Wheel[x;y;z][m],VehicleDynamics.Suspension.SuspensionFront.RelativePositionFront.Pos_Wheel[FL;FR][x;y;z][m].Pos_FL_Wheel[x;y;z][m],VehicleDynamics.Tire.r_Dyn_Tire[FL;FR;RL;RR][m]
  Bus Selector3 : BusSelector  OutputSignals=ESP_Switches
  Bus Selector4 : BusSelector  OutputSignals=ExternalModel.Reset_VehicleStates[0|1],ExternalModel.ECU_Commands[],ExternalModel.Pos_AccPedal[%],ExternalModel.Pos_BrakePedal[%]
  Engine_Topology_Switch : Subsystem
  HideBusFeedback : DataTypeConversion  SaturateOnIntegerOverflow=off  RndMeth=Floor
  HideBusFeedback1 : DataTypeConversion  SaturateOnIntegerOverflow=off  RndMeth=Floor
  Map_Inputs : Subsystem
  ModelDesk_MC_ID_SoftECU : ASM_Utils_lib/ModelDeskInterface/ModelDesk_MC  Tag=ASM_MAINCOMPONENT  Editable=off  MainComponent=SoftECU
  Mux1 : Mux
  OpenBrakeSoftECU : ASM_Utils_lib/Miscellaneous/OpenSystem  popupLibBlk=<select here>  popupTargetDemo=<select here>  Demosystem=BrakeHydraulics_SoftECU  variantLib=ASM_BrakeHydraulics_DemoSystems/SoftECU
  Soft_ECU_Brake : Subsystem  Tag=BrakeHydraulics_SoftECU
  ASMSignalBus : Outport  VectorParamsAs1DForOutWhenUnconnected=off
  Out : Outport  Port=2  VectorParamsAs1DForOutWhenUnconnected=off
  wires:
  UserInterface/1 -> Bus Selector3/1
  Map_Inputs/2(Sw_ASR[0Off|1On]) -> Soft_ECU_Brake/7(Sw_ASR[0Off|1On])
  Map_Inputs/1(Sw_ESP[0Off|1ABS|ESP]) -> Soft_ECU_Brake/6(Sw_ESP[0Off|1ABS|2ESP])
  HideBusFeedback1/1 -> Soft_ECU_Brake/3(Trq_Request_Extern[Nm])
  HideBusFeedback/1 -> Soft_ECU_Brake/1(State_Brake_Without_BrkPedal[0|1]), Soft_ECU_Brake/2(Enable_Trq_Extern[0|1])
  Bus Creator/1 -> Out/1
  Soft_ECU_Brake/2(Enable_p_Brake_Desired[0|1]) -> Bus Creator/1
  Soft_ECU_Brake/3(p_Brake_Desired[bar]) -> Bus Creator/2
  Soft_ECU_Brake/4(ECU_Mode[0None|1ABS|2ESP|3ASR]) -> Bus Creator/3
  Soft_ECU_Brake/5(Valves) -> Bus Creator/4
  Soft_ECU_Brake/6(Trq_Intervention) -> Bus Creator/5
  Bus Selector1/2 -> Brake_Topology_Switch/2(Trq_Brake_Request_Extern[Nm])  "<Trq_Brake_Request_Extern[Nm]>"
  Bus Selector1/1 -> Brake_Topology_Switch/1(Enable_Trq_Brake_Extern[0|1])  "<Enable_Trq_Brake_Extern[0|1]>"
  Interface_In/1 -> Bus Selector1/1, Bus Selector10/1, Bus Selector4/1
  Soft_ECU_Brake/1(ASMSignalBus) -> ASMSignalBus/1
  Bus Selector4/2 -> Map_Inputs/3(ECU_Commands[])  "<ECU_Commands[]>"
  Bus Selector4/1 -> Soft_ECU_Brake/5(Reset[]), Map_Inputs/1(Reset[0|1])  "<Reset_VehicleStates[0|1]>"
  Bus Selector4/3 -> Soft_ECU_Brake/17(Pos_AccPedal[%])  "<Pos_AccPedal[%]>"
  Bus Selector4/4 -> Soft_ECU_Brake/18(Pos_BrakePedal[%])  "<Pos_BrakePedal[%]>"
  Bus Selector3/1 -> Map_Inputs/2(Switches_ESP_User)  "<ESP_Switches>"
  Plant/1 -> Bus Selector2/1
  Bus Selector2/1 -> Mux1/1  "<Const_BrakeDiscFactor_FL[m3]>"
  Bus Selector2/2 -> Mux1/2  "<Const_BrakeDiscFactor_FR[m3]>"
  Bus Selector2/3 -> Mux1/3  "<Const_BrakeDiscFactor_RL[m3]>"
  Bus Selector2/4 -> Mux1/4  "<Const_BrakeDiscFactor_RR[m3]>"
  Mux1/1 -> Soft_ECU_Brake/4(Const_BrakeDiscFactor[FL;FR;RL;RR][m3])
  Bus Selector2/5 -> Soft_ECU_Brake/9(p_MasterBrakeCyl[bar])  "<p[bar]>"
  Bus Selector2/6 -> Soft_ECU_Brake/10(v_x_Vehicle_CoG[km|h])  "<v_x_Vehicle_CoG[km|h]>"
  Bus Selector2/7 -> Soft_ECU_Brake/11(v_y_Vehicle_CoG[km|h])  "<v_y_Vehicle_CoG[km|h]>"
  Bus Selector2/8 -> Soft_ECU_Brake/12(a_y_Vehicle_CoG[m|s2])  "<a_y_Vehicle_CoG[m|s2]>"
  Bus Selector2/9 -> Soft_ECU_Brake/13(YawRate_Vehicle_CoG[deg|s])  "<YawRate_Vehicle_CoG[deg|s]>"
  Bus Selector2/10 -> Soft_ECU_Brake/14(WheelSpeed[FL;FR;RL;RR][rad|s])  "<omega_Wheel[FL;FR;RL;RR][rad|s]>"
  Bus Selector2/11 -> Soft_ECU_Brake/15(Angle_SteeringWheel[deg])  "<Angle_SteeringWheel[deg]>"
  Bus Selector2/12 -> Soft_ECU_Brake/16(i_Steering_Mean[])  "<i_Steering_Mean[]>"
  Bus Selector2/13 -> Soft_ECU_Brake/19(Pos_RL_Wheel[x;y;z][m])  "<Pos_RL_Wheel[x;y;z][m]>"
  Bus Selector2/14 -> Soft_ECU_Brake/20(Pos_FL_Wheel[x;y;z][m])  "<Pos_FL_Wheel[x;y;z][m]>"
  Bus Selector2/15 -> Soft_ECU_Brake/21(r_Tire[m])  "<r_Dyn_Tire[FL;FR;RL;RR][m]>"
  Bus Selector1/3 -> Brake_Topology_Switch/3(Trq_Request_Brake[Nm])  "<Trq_Request_Brake[Nm]>"
  Brake_Topology_Switch/1(Enable_Trq_Extern[0|1]) -> HideBusFeedback/1
  Brake_Topology_Switch/2(Trq_Request_Extern[Nm]) -> HideBusFeedback1/1
  Engine_Topology_Switch/1(Trq[Nm]) -> Soft_ECU_Brake/8(Trq_Eff_Engine[Nm])
  Bus Selector10/1 -> Brake_Topology_Switch/4(Vehicle_Topology[-2|-1|0|2]), Engine_Topology_Switch/1(Vehicle_Topology[-2|-1|0|2])  "<Vehicle_Topology[-2|-1|0|2]>"
  Bus Selector10/2 -> Engine_Topology_Switch/2(Trq_Eff_Engine[Nm])  "<Trq_Eff_Engine[Nm]>"
  Bus Selector10/3 -> Engine_Topology_Switch/3(Trq_EM_Front[Nm])  "<Trq_EM_Front[Nm]>"

== system ASM_Traffic_A11/VehicleDynamics/Control/SoftECU_Steering ==
  note: -------------
  note: Control
  note: -------------
  note: -------------
  note: -------------
  note: Inport colors:
  note: User Interface
  note: Plant
  note: External Signals
  UserInterface : Inport
  Interface_In : Inport  Port=2
  Plant : Inport  Port=3
  Bus Creator : BusCreator  Inputs=1
  Bus Selector : BusSelector  OutputSignals=ExternalModel.Reset_VehicleStates[0|1],ExternalModel.Sw_Ignition[0Off|1On]
  Bus Selector1 : BusSelector  OutputSignals=VehicleDynamics.Steering.ForcesAndTorques.TrqSpring_SteeringColumn[Nm],VehicleDynamics.VehicleMovement.Velocities.Vehicle.Linear.v_Vehicle_CoG[x;y;z][km|h].v_x_Vehicle_CoG[km|h],VehicleDynamics.VehicleMovement.Velocities.Vehicle.Linear.v_Vehicle_CoG[x;y;z][km|h].v_y_Vehicle_CoG[km|h],VehicleDynamics.VehicleMovement.Velocities.Vehicle.Linear.v_Vehicle_CoG[x;y;z][km|h].v_z_Vehicle_CoG[km|h]
  ModelDesk_MC_ID_SoftECU : ASM_Utils_lib/ModelDeskInterface/ModelDesk_MC  Tag=ASM_MAINCOMPONENT  Editable=off  MainComponent=SoftECU
  Mux : Mux  Inputs=3
  SOFT_ECU_POWERSTEERING : ASM_VehicleDynamics_lib/SoftECU/SoftECU_Steering/SOFT_ECU_POWERSTEERING  Tag=ASM_SUBCOMPONENT  Const_t_PowerSteering=MDL.SoftECU.SoftECUPowerSteering.Const_t_PowerSteering  Map_Trq_PowerSteering=MDL.SoftECU.SoftECUPowerSteering.Map_Trq_PowerSteering  StepSize=SIM.StepSize  ASMProperties=struct('Name','SOFT_ECU_POWERSTEERING','Version','3.0','Library','ASM_VehicleDynamics_lib')  ASMInstanceName=soft_ecu_powersteering  ASMInstanceID=1
  Terminator_1 : Terminator
  ASMSignalBus : Outport  VectorParamsAs1DForOutWhenUnconnected=off
  Out : Outport  Port=2  VectorParamsAs1DForOutWhenUnconnected=off
  wires:
  UserInterface/1 -> Terminator_1/1
  Interface_In/1 -> Bus Selector/1
  Plant/1 -> Bus Selector1/1
  Bus Selector/2 -> SOFT_ECU_POWERSTEERING/4  "<Sw_Ignition[0Off|1On]>"
  Bus Creator/1 -> Out/1
  SOFT_ECU_POWERSTEERING/2 -> Bus Creator/1  "Trq_PowerSteering[Nm]"
  Bus Selector/1 -> SOFT_ECU_POWERSTEERING/2  "<Reset_VehicleStates[0|1]>"
  Mux/1 -> SOFT_ECU_POWERSTEERING/3
  Bus Selector1/1 -> SOFT_ECU_POWERSTEERING/1  "<TrqSpring_SteeringColumn[Nm]>"
  SOFT_ECU_POWERSTEERING/1 -> ASMSignalBus/1
  Bus Selector1/4 -> Mux/3  "<v_z_Vehicle_CoG[km|h]>"
  Bus Selector1/3 -> Mux/2  "<v_y_Vehicle_CoG[km|h]>"
  Bus Selector1/2 -> Mux/1  "<v_x_Vehicle_CoG[km|h]>"

== system ASM_Traffic_A11/VehicleDynamics/Control/Sw_ECU_Brake_Signals ==
  SoftECU : Inport
  ExternalECU : Inport  Port=2
  Bus Creator : BusCreator  Inputs=13
  Bus Creator1 : BusCreator  Inputs=2
  Bus Creator2 : BusCreator  Inputs=4
  Bus Creator3 : BusCreator  Inputs=6
  Bus Creator7 : BusCreator  Inputs=1
  Bus Selector2 : BusSelector  OutputSignals=ExternalECU.Brake.Enable_p_Brake_Desired[0|1],ExternalECU.Brake.p_Brake_Desired[bar],ExternalECU.Brake.Enable_TrqDecrease_Fast_ESP[0|1],ExternalECU.Brake.Trq_DecreaseRequest_Fast_ESP[Nm],ExternalECU.Brake.Enable_TrqDecrease_Slow_ESP[0|1],ExternalECU.Brake.Trq_DecreaseRequest_Slow_ESP[Nm],ExternalECU.Brake.Enable_TrqIncrease_ESP[0|1],ExternalECU.Brake.Trq_IncreaseRequest_ESP[Nm],ExternalECU.Brake.Ctrl_InletValve_FL[0_1],ExternalECU.Brake.Ctrl_InletValve_FR[0_1],ExternalECU.Brake.Ctrl_InletValve_RL[0_1],ExternalECU.Brake.Ctrl_InletValve_RR[0_1],ExternalECU.Brake.Ctrl_OutletValve_FL[0_1],ExternalECU.Brake.Ctrl_OutletValve_FR[0_1],ExternalECU.Brake.Ctrl_OutletValve_RL[0_1],ExternalECU.Brake.Ctrl_OutletValve_RR[0_1],ExternalECU.Brake.Ctrl_PreChargeValve_1[0_1],ExternalECU.Brake.Ctrl_PreChargeValve_2[0_1],ExternalECU.Brake.Ctrl_ChangeOverValve_1[0_1],ExternalECU.Brake.Ctrl_ChangeOverValve_2[0_1],ExternalECU.Brake.Ctrl_HydPump[0_1],ExternalECU.Brake.ECU_ESP_Mode[0None|1ABS|2ESP|3ASR]
  Bus Selector3 : BusSelector  OutputSignals=Enable_p_Brake_Desired[0|1],p_Brake_Desired[bar],Trq_Intervention.Enable_TrqDecrease_Fast_ESP[0|1],Trq_Intervention.Trq_DecreaseRequest_Fast_ESP[Nm],Trq_Intervention.Enable_TrqDecrease_Slow_ESP[0|1],Trq_Intervention.Trq_DecreaseRequest_Slow_ESP[Nm],Trq_Intervention.Enable_TrqIncrease_ESP[0|1],Trq_Intervention.Trq_IncreaseRequest_ESP[Nm],Valves.Ctrl_InletValve_FL[0_1],Valves.Ctrl_InletValve_FR[0_1],Valves.Ctrl_InletValve_RL[0_1],Valves.Ctrl_InletValve_RR[0_1],Valves.Ctrl_OutletValve_FL[0_1],Valves.Ctrl_OutletValve_FR[0_1],Valves.Ctrl_OutletValve_RL[0_1],Valves.Ctrl_OutletValve_RR[0_1],Valves.Ctrl_PreChargeValve_1[0_1],Valves.Ctrl_PreChargeValve_2[0_1],Valves.Ctrl_ChangeOverValve_1[0_1],Valves.Ctrl_ChangeOverValve_2[0_1],Valves.Ctrl_HydPump[0_1],ECU_Mode[0None|1ABS|2ESP|3ASR]
  Ctrl_ChangeOverValve_1[0_1] : Subsystem
  Ctrl_ChangeOverValve_2[0_1] : Subsystem
  Ctrl_HydPump[0_1] : Subsystem
  Ctrl_InletValve_FL[0_1] : Subsystem
  Ctrl_InletValve_FR[0_1] : Subsystem
  Ctrl_InletValve_RL[0_1] : Subsystem
  Ctrl_InletValve_RR[0_1] : Subsystem
  Ctrl_OutletValve_FL[0_1] : Subsystem
  Ctrl_OutletValve_FR[0_1] : Subsystem
  Ctrl_OutletValve_RL[0_1] : Subsystem
  Ctrl_OutletValve_RR[0_1] : Subsystem
  Ctrl_PreChargeValve_1[0_1] : Subsystem
  Ctrl_PreChargeValve_2[0_1] : Subsystem
  ECU_ESP_Mode[0None|1ABS|2ESP|3ASR] : Subsystem
  Enable_TrqDecrease_Fast_ESP[0|1] : Subsystem
  Enable_TrqDecrease_Slow_ESP[0|1] : Subsystem
  Enable_TrqIncrease_ESP[0|1] : Subsystem
  Enable_p_Brake_Desired[0|1] : Subsystem
  Trq_DecreaseRequest_Fast_ESP[Nm] : Subsystem
  Trq_DecreaseRequest_Slow_ESP[Nm] : Subsystem
  Trq_IncreaseRequest_ESP[Nm] : Subsystem
  p_Brake_Desired[bar] : Subsystem
  ECU_Signals : Outport  VectorParamsAs1DForOutWhenUnconnected=off
  wires:
  SoftECU/1 -> Bus Selector3/1
  Bus Selector2/22 -> ECU_ESP_Mode[0None|1ABS|2ESP|3ASR]/2(RealECU)  "<ECU_ESP_Mode[0None|1ABS|2ESP|3ASR]>"
  Bus Selector2/21 -> Ctrl_HydPump[0_1]/2(RealECU)  "<Ctrl_HydPump[0_1]>"
  Bus Selector2/20 -> Ctrl_ChangeOverValve_2[0_1]/2(RealECU)  "<Ctrl_ChangeOverValve_2[0_1]>"
  Bus Selector2/19 -> Ctrl_ChangeOverValve_1[0_1]/2(RealECU)  "<Ctrl_ChangeOverValve_1[0_1]>"
  Bus Selector2/18 -> Ctrl_PreChargeValve_2[0_1]/2(RealECU)  "<Ctrl_PreChargeValve_2[0_1]>"
  Bus Selector2/17 -> Ctrl_PreChargeValve_1[0_1]/2(RealECU)  "<Ctrl_PreChargeValve_1[0_1]>"
  Bus Selector2/16 -> Ctrl_OutletValve_RR[0_1]/2(RealECU)  "<Ctrl_OutletValve_RR[0_1]>"
  Bus Selector2/15 -> Ctrl_OutletValve_RL[0_1]/2(RealECU)  "<Ctrl_OutletValve_RL[0_1]>"
  Bus Selector2/14 -> Ctrl_OutletValve_FR[0_1]/2(RealECU)  "<Ctrl_OutletValve_FR[0_1]>"
  Bus Selector2/13 -> Ctrl_OutletValve_FL[0_1]/2(RealECU)  "<Ctrl_OutletValve_FL[0_1]>"
  Bus Selector2/12 -> Ctrl_InletValve_RR[0_1]/2(RealECU)  "<Ctrl_InletValve_RR[0_1]>"
  Bus Selector2/11 -> Ctrl_InletValve_RL[0_1]/2(RealECU)  "<Ctrl_InletValve_RL[0_1]>"
  Bus Selector2/10 -> Ctrl_InletValve_FR[0_1]/2(RealECU)  "<Ctrl_InletValve_FR[0_1]>"
  Bus Selector2/9 -> Ctrl_InletValve_FL[0_1]/2(RealECU)  "<Ctrl_InletValve_FL[0_1]>"
  Bus Selector2/8 -> Trq_IncreaseRequest_ESP[Nm]/2(RealECU)  "<Trq_IncreaseRequest_ESP[Nm]>"
  Bus Selector2/7 -> Enable_TrqIncrease_ESP[0|1]/2(RealECU)  "<Enable_TrqIncrease_ESP[0|1]>"
  Bus Selector2/6 -> Trq_DecreaseRequest_Slow_ESP[Nm]/2(RealECU)  "<Trq_DecreaseRequest_Slow_ESP[Nm]>"
  Bus Selector2/5 -> Enable_TrqDecrease_Slow_ESP[0|1]/2(RealECU)  "<Enable_TrqDecrease_Slow_ESP[0|1]>"
  Bus Selector2/4 -> Trq_DecreaseRequest_Fast_ESP[Nm]/2(RealECU)  "<Trq_DecreaseRequest_Fast_ESP[Nm]>"
  Bus Selector2/3 -> Enable_TrqDecrease_Fast_ESP[0|1]/2(RealECU)  "<Enable_TrqDecrease_Fast_ESP[0|1]>"
  Bus Selector2/2 -> p_Brake_Desired[bar]/2(RealECU)  "<p_Brake_Desired[bar]>"
  Bus Selector2/1 -> Enable_p_Brake_Desired[0|1]/2(RealECU)  "<Enable_p_Brake_Desired[0|1]>"
  ExternalECU/1 -> Bus Selector2/1
  Ctrl_InletValve_FL[0_1]/1(Ctrl_InletValve_FL[0_1]) -> Bus Creator/1  "Ctrl_InletValve_FL[0_1]"
  Ctrl_InletValve_FR[0_1]/1(Ctrl_InletValve_FR[0_1]) -> Bus Creator/2  "Ctrl_InletValve_FR[0_1]"
  Ctrl_InletValve_RL[0_1]/1(Ctrl_InletValve_RL[0_1]) -> Bus Creator/3  "Ctrl_InletValve_RL[0_1]"
  Ctrl_InletValve_RR[0_1]/1(Ctrl_InletValve_RR[0_1]) -> Bus Creator/4  "Ctrl_InletValve_RR[0_1]"
  Ctrl_OutletValve_FL[0_1]/1(Ctrl_OutletValve_FL[0_1]) -> Bus Creator/5  "Ctrl_OutletValve_FL[0_1]"
  Ctrl_OutletValve_FR[0_1]/1(Ctrl_OutletValve_FR[0_1]) -> Bus Creator/6  "Ctrl_OutletValve_FR[0_1]"
  Ctrl_OutletValve_RL[0_1]/1(Ctrl_OutletValve_RL[0_1]) -> Bus Creator/7  "Ctrl_OutletValve_RL[0_1]"
  Ctrl_OutletValve_RR[0_1]/1(Ctrl_OutletValve_RR[0_1]) -> Bus Creator/8  "Ctrl_OutletValve_RR[0_1]"
  Ctrl_PreChargeValve_1[0_1]/1(Ctrl_PreChargeValve_1[0_1]) -> Bus Creator/9  "Ctrl_PreChargeValve_1[0_1]"
  Ctrl_PreChargeValve_2[0_1]/1(Ctrl_PreChargeValve_2[0_1]) -> Bus Creator/10  "Ctrl_PreChargeValve_2[0_1]"
  Ctrl_ChangeOverValve_1[0_1]/1(Ctrl_ChangeOverValve_1[0_1]) -> Bus Creator/11  "Ctrl_ChangeOverValve_1[0_1]"
  Ctrl_ChangeOverValve_2[0_1]/1(Ctrl_ChangeOverValve_2[0_1]) -> Bus Creator/12  "Ctrl_ChangeOverValve_2[0_1]"
  Bus Creator/1 -> Bus Creator2/3  "Valves"
  Ctrl_HydPump[0_1]/1(Ctrl_HydPump[0_1]) -> Bus Creator/13  "Ctrl_HydPump[0_1]"
  Enable_TrqDecrease_Fast_ESP[0|1]/1(Enable_TrqDecrease_Fast[0|1]) -> Bus Creator3/1  "Enable_TrqDecrease_Fast_ESP[0|1]"
  Trq_DecreaseRequest_Slow_ESP[Nm]/1(Trq_DecreaseRequest_Slow[Nm]) -> Bus Creator3/4  "Trq_DecreaseRequest_Slow_ESP[Nm]"
  Enable_TrqIncrease_ESP[0|1]/1(Enable_TrqIncrease[0|1]) -> Bus Creator3/5  "Enable_TrqIncrease_ESP[0|1]"
  Trq_IncreaseRequest_ESP[Nm]/1(Trq_IncreaseRequest[Nm]) -> Bus Creator3/6  "Trq_IncreaseRequest_ESP[Nm]"
  Trq_DecreaseRequest_Fast_ESP[Nm]/1(Trq_DecreaseRequest_Fast[Nm]) -> Bus Creator3/2  "Trq_DecreaseRequest_Fast_ESP[Nm]"
  Bus Creator3/1 -> Bus Creator2/2  "ESP_Trq_Intervention"
  Enable_TrqDecrease_Slow_ESP[0|1]/1(Enable_TrqDecrease_Slow[0|1]) -> Bus Creator3/3  "Enable_TrqDecrease_Slow_ESP[0|1]"
  Bus Selector3/1 -> Enable_p_Brake_Desired[0|1]/1(SoftECU)  "<Enable_p_Brake_Desired[0|1]>"
  Bus Selector3/2 -> p_Brake_Desired[bar]/1(SoftECU)  "<p_Brake_Desired[bar]>"
  Bus Selector3/3 -> Enable_TrqDecrease_Fast_ESP[0|1]/1(SoftECU)  "<Enable_TrqDecrease_Fast_ESP[0|1]>"
  Bus Selector3/4 -> Trq_DecreaseRequest_Fast_ESP[Nm]/1(SoftECU)  "<Trq_DecreaseRequest_Fast_ESP[Nm]>"
  Enable_p_Brake_Desired[0|1]/1(Enable_p_Brake_Desired[0|1]) -> Bus Creator1/1  "Enable_p_Brake_Desired[0|1]"
  p_Brake_Desired[bar]/1(p_Brake_Desired[bar]) -> Bus Creator1/2  "p_Brake_Desired[bar]"
  Bus Creator1/1 -> Bus Creator2/1  "DesiredPressure"
  ECU_ESP_Mode[0None|1ABS|2ESP|3ASR]/1(ECU_ESP_Mode[0None|1ABS|2ESP|3ASR]) -> Bus Creator7/1  "ECU_ESP_Mode[0None|1ABS|2ESP|3ASR]"
  Bus Creator7/1 -> Bus Creator2/4  "ECU_Mode"
  Bus Creator2/1 -> ECU_Signals/1  "ECU_Brake"
  Bus Selector3/9 -> Ctrl_InletValve_FL[0_1]/1(SoftECU)  "<Ctrl_InletValve_FL[0_1]>"
  Bus Selector3/10 -> Ctrl_InletValve_FR[0_1]/1(SoftECU)  "<Ctrl_InletValve_FR[0_1]>"
  Bus Selector3/11 -> Ctrl_InletValve_RL[0_1]/1(SoftECU)  "<Ctrl_InletValve_RL[0_1]>"
  Bus Selector3/12 -> Ctrl_InletValve_RR[0_1]/1(SoftECU)  "<Ctrl_InletValve_RR[0_1]>"
  Bus Selector3/13 -> Ctrl_OutletValve_FL[0_1]/1(SoftECU)  "<Ctrl_OutletValve_FL[0_1]>"
  Bus Selector3/14 -> Ctrl_OutletValve_FR[0_1]/1(SoftECU)  "<Ctrl_OutletValve_FR[0_1]>"
  Bus Selector3/15 -> Ctrl_OutletValve_RL[0_1]/1(SoftECU)  "<Ctrl_OutletValve_RL[0_1]>"
  Bus Selector3/16 -> Ctrl_OutletValve_RR[0_1]/1(SoftECU)  "<Ctrl_OutletValve_RR[0_1]>"
  Bus Selector3/17 -> Ctrl_PreChargeValve_1[0_1]/1(SoftECU)  "<Ctrl_PreChargeValve_1[0_1]>"
  Bus Selector3/18 -> Ctrl_PreChargeValve_2[0_1]/1(SoftECU)  "<Ctrl_PreChargeValve_2[0_1]>"
  Bus Selector3/19 -> Ctrl_ChangeOverValve_1[0_1]/1(SoftECU)  "<Ctrl_ChangeOverValve_1[0_1]>"
  Bus Selector3/20 -> Ctrl_ChangeOverValve_2[0_1]/1(SoftECU)  "<Ctrl_ChangeOverValve_2[0_1]>"
  Bus Selector3/21 -> Ctrl_HydPump[0_1]/1(SoftECU)  "<Ctrl_HydPump[0_1]>"
  Bus Selector3/22 -> ECU_ESP_Mode[0None|1ABS|2ESP|3ASR]/1(SoftECU)  "<ECU_Mode[0None|1ABS|2ESP|3ASR]>"
  Bus Selector3/5 -> Enable_TrqDecrease_Slow_ESP[0|1]/1(SoftECU)  "<Enable_TrqDecrease_Slow_ESP[0|1]>"
  Bus Selector3/6 -> Trq_DecreaseRequest_Slow_ESP[Nm]/1(SoftECU)  "<Trq_DecreaseRequest_Slow_ESP[Nm]>"
  Bus Selector3/7 -> Enable_TrqIncrease_ESP[0|1]/1(SoftECU)  "<Enable_TrqIncrease_ESP[0|1]>"
  Bus Selector3/8 -> Trq_IncreaseRequest_ESP[Nm]/1(SoftECU)  "<Trq_IncreaseRequest_ESP[Nm]>"

== system ASM_Traffic_A11/VehicleDynamics/Control/Sw_ECU_Steering_Signals ==
  SoftECU : Inport
  ExternalECU : Inport  Port=2
  Bus Creator6 : BusCreator  Inputs=1
  Bus Selector1 : BusSelector  OutputSignals=ExternalECU.Steering.Trq_PowerSteering[Nm]
  Bus Selector4 : BusSelector  OutputSignals=Trq_PowerSteering[Nm]
  Trq_PowerSteering[Nm] : Subsystem
  ECU_Signals : Outport  VectorParamsAs1DForOutWhenUnconnected=off
  wires:
  Bus Selector1/1 -> Trq_PowerSteering[Nm]/2(RealECU)  "<Trq_PowerSteering[Nm]>"
  Bus Creator6/1 -> ECU_Signals/1  "ECU_Steering"
  Bus Selector4/1 -> Trq_PowerSteering[Nm]/1(SoftECU)  "<Trq_PowerSteering[Nm]>"
  SoftECU/1 -> Bus Selector4/1
  Trq_PowerSteering[Nm]/1(Trq_PowerSteering[Nm]) -> Bus Creator6/1  "Trq_PowerSteering[Nm]"
  ExternalECU/1 -> Bus Selector1/1

== system ASM_Traffic_A11/VehicleDynamics/Control/UserInterface ==
  note: VehicleDynamics Control
  In : Inport
  ASMSignalBus_Control : Subsystem
  DISP_Control : Subsystem
  PAR_Control : Subsystem
  Out : Outport  VectorParamsAs1DForOutWhenUnconnected=off
  wires:
  In/1 -> ASMSignalBus_Control/1(In), DISP_Control/1(In)
  PAR_Control/1(Out) -> Out/1
